simulink model "Y3Tiltrotor_sim3_INDI"  (R2025a)
settings: Solver=ode4  StartTime=0.0  StopTime=70  FixedStep=uavParam.sampleTime  RelTol=1e-3
PreLoadFcn:
  | filepath  = fileparts(get_param(bdroot, 'FileName'))
  | cd(filepath);
InitFcn:
  | Init_sim_INDI;
values from neighbouring files (symbols this model uses):
  control = struct    [Init_sim_INDI.m]
  env = struct    [InitData.m]
  flightState = struct    [Init_sim_INDI.m]
  FWSpeed0 = 15    [Init_sim_INDI.m]
  k_lpf_p = 50    [Init_sim_INDI.m]
  k_lpf_q = 80    [Init_sim_INDI.m]
  k_lpf_r = 5    [Init_sim_INDI.m]
  k_lpf_u = 10    [Init_sim_INDI.m]
  k_lpf_v = 1    [Init_sim_INDI.m]
  k_lpf_w = 50    [Init_sim_INDI.m]
  k_p = 5    [Init_sim_INDI.m]
  k_q = 20    [Init_sim_INDI.m]
  k_r = 1.5    [Init_sim_INDI.m]
  k_u = 0.5    [Init_sim_INDI.m]
  k_v = 0.5    [Init_sim_INDI.m]
  k_w = 2    [Init_sim_INDI.m]
  uavParam = struct    [InitData.m]
undefined symbols (not defined in the file or in its folder): ControlSampleTime, F, Light, MIL, Newton, Raphson
libraries: slpidlib x28, SignalEditorBlockLib x12, simulink x6, aerolibtransform2 x3, sharedtransform x3, robotcorelib x3, matrix_library x3, aerolibasang x2, aerolibutil x2, aerolibwind2 x2, shared6dof x1, aerolibatmos2 x1
(part 6 of 7)

== system Y3Tiltrotor_sim3_INDI/Y3 Tiltrotor Aircraft Model/Subsystem/Aerodynamic Forces and Moments/Compute Body Frame Aerodynamic Forces and Moments/Aerodynamic Forces and Moment Calculations/Subsystem1 ==
  AirData : Inport
  M_w : Inport  Port=2
  Bus Selector : BusSelector  OutputSignals=alpha,beta
  Direction Cosine Matrix Body to Wind : aerolibtransform2/Direction Cosine Matrix Body to Wind
  Mux1 : Mux  Inputs=2
  Product2 : Product  Multiplication=Matrix(*)  RndMeth=Zero
  Reshape1 : Reshape  OutputDimensionality=Column vector (2-D)
  Reshape2 : Reshape
  Transpose : Math  Operator=transpose  SignedPower=on
  M_b : Outport
  wires:
  AirData/1 -> Bus Selector/1
  Bus Selector/2 -> Mux1/2  "<beta>"
  Bus Selector/1 -> Mux1/1  "<alpha>"
  Direction Cosine Matrix Body to Wind/1 -> Transpose/1
  Reshape2/1 -> M_b/1
  Reshape1/1 -> Product2/2
  M_w/1 -> Reshape1/1
  Mux1/1 -> Direction Cosine Matrix Body to Wind/1
  Product2/1 -> Reshape2/1
  Transpose/1 -> Product2/1

== system Y3Tiltrotor_sim3_INDI/Y3 Tiltrotor Aircraft Model/Subsystem/Aerodynamic Forces and Moments/Compute Body Frame Aerodynamic Forces and Moments/Wind frame F& M/Lateral Channel ==
  note: 飞机没有尾翼，不需要考虑方向舵的影响，固定翼模态下做偏航运动时通过两个螺旋桨的推力差动来实现；其造成的侧力与偏航力矩在旋翼建模部分计算。
  beta : Inport
  dA : Inport  Port=2
  Bus Creator : BusCreator  Inputs=3
  CY : Subsystem
  Cl : Subsystem
  Cn : Subsystem
  Saturation2 : Saturate  UpperLimit=pi/2  LowerLimit=-pi/2
  固定翼模态使用 : Saturate  UpperLimit=41.5*pi/80  LowerLimit=-41.5*pi/80
  旋翼模态使用 : Saturate  UpperLimit=90*pi/80  LowerLimit=-90*pi/80
  Lateral : Outport  VectorParamsAs1DForOutWhenUnconnected=off
  wires:
  Cl/1(Cl) -> Bus Creator/2  "Cl"
  Cn/1(Cn) -> Bus Creator/3  "Cn"
  CY/1(CY) -> Bus Creator/1  "CY"
  Bus Creator/1 -> Lateral/1
  beta/1 -> 旋翼模态使用/1
  dA/1 -> Saturation2/1
  旋翼模态使用/1 -> Cn/1(beta), Cl/1(beta), CY/1(beta)
  Saturation2/1 -> Cn/2(dA), Cl/2(dA)

== system Y3Tiltrotor_sim3_INDI/Y3 Tiltrotor Aircraft Model/Subsystem/Aerodynamic Forces and Moments/Compute Body Frame Aerodynamic Forces and Moments/Wind frame F& M/Longitudinal Channel ==
  alpha : Inport
  dE : Inport  Port=2
  dA : Inport  Port=3
  Bus Creator : BusCreator  Inputs=3
  CD : Subsystem
  CL : Subsystem
  Cm : Subsystem
  Saturation1 : Saturate  UpperLimit=pi/2  LowerLimit=-pi/2
  Saturation2 : Saturate  UpperLimit=pi/2  LowerLimit=-pi/2
  固定翼模态使用 : Saturate  UpperLimit=18.4*pi/180  LowerLimit=-15*pi/180  LinearizeAsGain=off  ZeroCross=off
  旋翼模态使用 : Saturate  UpperLimit=90*pi/80  LowerLimit=-90*pi/80
  Longitudinal : Outport  VectorParamsAs1DForOutWhenUnconnected=off
  wires:
  Bus Creator/1 -> Longitudinal/1
  Cm/1(Cm) -> Bus Creator/3  "Cm"
  CL/1(CL) -> Bus Creator/2  "CL"
  CD/1(CD) -> Bus Creator/1  "CD"
  alpha/1 -> 旋翼模态使用/1
  dE/1 -> Saturation1/1
  Saturation1/1 -> Cm/2(dE), CL/2(dE), CD/2(dE)
  旋翼模态使用/1 -> Cm/1(alpha), CL/1(alpha), CD/1(alpha)
  dA/1 -> Saturation2/1
  Saturation2/1 -> CD/3(dA)

== system Y3Tiltrotor_sim3_INDI/Y3 Tiltrotor Aircraft Model/Subsystem/Aerodynamic Forces and Moments/Compute Body Frame Aerodynamic Forces and Moments/Wind frame F& M/Route coefficients ==
  Lateral : Inport
  Longitudinal : Inport  Port=2
  Bus Selector : BusSelector  OutputSignals=CY,Cl,Cn
  Bus Selector3 : BusSelector  OutputSignals=CD,CL,Cm
  <CD> : Outport
  <CY> : Outport  Port=2
  <CL> : Outport  Port=3
  <Cl> : Outport  Port=4
  <Cm> : Outport  Port=5
  <Cn> : Outport  Port=6
  wires:
  Bus Selector3/2 -> <CL>/1  "<CL>"
  Bus Selector/3 -> <Cn>/1  "<Cn>"
  Bus Selector/2 -> <Cl>/1  "<Cl>"
  Lateral/1 -> Bus Selector/1
  Bus Selector3/3 -> <Cm>/1  "<Cm>"
  Bus Selector3/1 -> <CD>/1  "<CD>"
  Longitudinal/1 -> Bus Selector3/1
  Bus Selector/1 -> <CY>/1  "<CY>"

== system Y3Tiltrotor_sim3_INDI/Subsystem/固定翼模态/高度-速度控制/定速模式/Subsystem1/Subsystem/InputConditioning_altitude ==
  Manual Vz_d : Inport
  Xe : Inport  Port=2
  Action Port : ActionPort  ActionPortLabel=case [ 1 ]:
  MATLAB Function : MATLAB Function  TreatAsAtomicUnit=on
  Selector : Selector  InputPortWidth=3  IndexOptions=Index vector (dialog)  Indices=3  OutputSizes=1
  manual_vz_cmd : Outport  VectorParamsAs1DForOutWhenUnconnected=off
  wires:
  MATLAB Function/1(vz_cmd) -> manual_vz_cmd/1
  Manual Vz_d/1 -> MATLAB Function/1(u)
  Selector/1 -> MATLAB Function/2(z_e)
  Xe/1 -> Selector/1

== system Y3Tiltrotor_sim3_INDI/Subsystem/固定翼模态/高度-速度控制/定速模式/Subsystem1/Subsystem/Subsystem ==
  Navigation Z : Inport
  Xe : Inport  Port=2
  Action Port : ActionPort  ActionPortLabel=case [ 0 ]:
  PID Controller1 : slpidlib/PID Controller  Controller=PID  Form=Parallel  TimeDomain=Continuous-time  UseExternalTs=off  SampleTime=ControlSampleTime  IntegratorMethod=Forward Euler  FilterMethod=Forward Euler  ControllerParametersSource=internal  P=control.FW.alt_P  I=control.FW.alt_I  UseKiTs=off  D=control.FW.alt_D  UseExternalDerivativeSource=off  N=100  UseFilter=on  TunerSelectOption=Transfer Function Based (PID Tuner App)  InitialConditionSource=internal  InitialConditionForIntegrator=0  InitialConditionForFilter=0  DifferentiatorICPrevScaledInput=0  ExternalReset=none  TrackingMode=off  Kt=1  LimitOutput=on  SatLimitsSource=internal  UpperSaturationLimit=control.maxClimbRate  LowerSaturationLimit=control.maxDescendRate  LinearizeAsGain=on  AntiWindupMode=clamping  Kb=1  LimitIntegrator=off  UpperIntegratorSaturationLimit=inf  LowerIntegratorSaturationLimit=-inf  POutMin=[]  POutMax=[]  IOutMin=[]  IOutMax=[]  DOutMin=[]  DOutMax=[]  NOutMin=[]  NOutMax=[]  SumOutMin=[]  SumOutMax=[]  SaturationOutMin=[]  SaturationOutMax=[]  PParamMin=[]  PParamMax=[]  IParamMin=[]  IParamMax=[]  DParamMin=[]  DParamMax=[]  NParamMin=[]  NParamMax=[]  KbParamMin=[]  KbParamMax=[]  KtParamMin=[]  KtParamMax=[]  KbOutMin=[]  KbOutMax=[]  KtOutMin=[]  KtOutMax=[]  IntegratorOutMin=[]  IntegratorOutMax=[]  FilterOutMin=[]  FilterOutMax=[]  SumI1OutMin=[]  SumI1OutMax=[]  SumI2OutMin=[]  SumI2OutMax=[]  SumI3OutMin=[]  SumI3OutMax=[]  SumI4OutMin=[]  SumI4OutMax=[]  SumDOutMin=[]  SumDOutMax=[]  DifferentiatorOutMin=[]  DifferentiatorOutMax=[]  FilterDiffOutCoefMin=[]  FilterDiffOutCoefMax=[]  ReciprocalOutMin=[]  ReciprocalOutMax=[]  SumDenOutMin=[]  SumDenOutMax=[]  SumNumOutMin=[]  SumNumOutMax=[]  DivideOutMin=[]  DivideOutMax=[]  UdiffTsProdOutMin=[]  UdiffTsProdOutMax=[]  NTsProdOutMin=[]  NTsProdOutMax=[]  UintegralTsProdOutMin=[]  UintegralTsProdOutMax=[]  UngainTsProdOutMin=[]  UngainTsProdOutMax=[]  ClampingZeroOutDataTypeStr=Inherit: Inherit via back propagation  ClampingZeroOutMin=[]  ClampingZeroOutMax=[]  FilterDenConstantOutDataTypeStr=Inherit: Inherit via back propagation  FilterDenConstantOutMin=[]  FilterDenConstantOutMax=[]  PCopyOutDataTypeStr=Inherit: Inherit via back propagation  PCopyOutMin=[]  PCopyOutMax=[]  NCopyOutDataTypeStr=Inherit: Inherit via back propagation  NCopyOutMin=[]  NCopyOutMax=[]  IntegratorContinuousStateAttributes=''  IntegratorStateMustResolveToSignalObject=off  IntegratorRTWStateStorageClass=Auto  FilterContinuousStateAttributes=''  FilterStateMustResolveToSignalObject=off  FilterRTWStateStorageClass=Auto  ParallelPVariant=InternalParameters  IdealPVariant=Disabled  IVariant=InternalParameters  DVariant=InternalParameters  IntegratorVariant=Continuous  SatVariant=Enabled  AWVariant=ContClampingParallel  PCopyVariant=Disabled  TRVariant=Disabled  FdbkBlocksVariant=Forward  IdealPFdbkVariant=Disabled  SatFdbkVariant=Disabled  DerivativeFilterVariant=ContFilter  NVariant=InternalParameters  NCopyVariant=Disabled  FilterICVariant=InternalICsFilter  IntegratorICVariant=InternalICs  ExternalResetVariant=Disabled  TRSumVariant=Passthrough  SumFdbkVariant=Disabled  SumVariant=Sum_PID  TsampFilterVariant=InternalTs  TsampNgainVariant=Passthrough  TsampIntegralVariant=Disabled_SignalSpec  ExternalSaturationOutDataTypeStr=Inherit: Same as second input  DerivativeSourceVariant=ErrorSignal  PreIntVariant=InternalPreInt
  Selector : Selector  InputPortWidth=3  IndexOptions=Index vector (dialog)  Indices=3  OutputSizes=1
  Sum : Sum  Inputs=|+-
  Unary Minus : UnaryMinus
  PID_vz_cmd : Outport
  wires:
  Unary Minus/1 -> Sum/2
  Selector/1 -> Unary Minus/1
  Xe/1 -> Selector/1
  Sum/1 -> PID Controller1/1
  PID Controller1/1 -> PID_vz_cmd/1
  Navigation Z/1 -> Sum/1

== system Y3Tiltrotor_sim3_INDI/Y3 Tiltrotor Aircraft Model/Subsystem/Aerodynamic Forces and Moments/Compute Body Frame Aerodynamic Forces and Moments/Wind frame F& M/Lateral Channel/CY ==
  beta : Inport
  CY(beta) : MATLAB Function  TreatAsAtomicUnit=on
  Gain : Gain  Gain=180/pi
  CY : Outport  VectorParamsAs1DForOutWhenUnconnected=off
  wires:
  CY(beta)/1(CY_beta) -> CY/1
  beta/1 -> Gain/1
  Gain/1 -> CY(beta)/1(beta)

== system Y3Tiltrotor_sim3_INDI/Y3 Tiltrotor Aircraft Model/Subsystem/Aerodynamic Forces and Moments/Compute Body Frame Aerodynamic Forces and Moments/Wind frame F& M/Lateral Channel/Cl ==
  beta : Inport
  dA : Inport  Port=2
  Cl(beta) : MATLAB Function  TreatAsAtomicUnit=on
  Cl(delta_a) : MATLAB Function  TreatAsAtomicUnit=on
  Gain : Gain  Gain=180/pi
  Gain1 : Gain  Gain=180/pi
  Gain2 : Gain
  Sum : Sum  Inputs=|++
  Cl : Outport  VectorParamsAs1DForOutWhenUnconnected=off
  wires:
  Gain/1 -> Cl(beta)/1(beta)
  beta/1 -> Gain/1
  dA/1 -> Gain1/1
  Sum/1 -> Gain2/1
  Gain1/1 -> Cl(delta_a)/1(delta_a)
  Cl(delta_a)/1(Cl1_delta_a) -> Sum/2
  Cl(beta)/1(Cl1_beta) -> Sum/1
  Gain2/1 -> Cl/1

== system Y3Tiltrotor_sim3_INDI/Y3 Tiltrotor Aircraft Model/Subsystem/Aerodynamic Forces and Moments/Compute Body Frame Aerodynamic Forces and Moments/Wind frame F& M/Lateral Channel/Cn ==
  beta : Inport
  dA : Inport  Port=2
  Cn(beta) : MATLAB Function  TreatAsAtomicUnit=on
  Cn(delta_a) : MATLAB Function  TreatAsAtomicUnit=on
  Gain : Gain  Gain=180/pi
  Gain1 : Gain  Gain=180/pi
  Gain2 : Gain
  Sum : Sum  Inputs=|++
  Cn : Outport  VectorParamsAs1DForOutWhenUnconnected=off
  wires:
  dA/1 -> Gain1/1
  beta/1 -> Gain/1
  Gain/1 -> Cn(beta)/1(beta)
  Sum/1 -> Gain2/1
  Cn(beta)/1(Cn_beta) -> Sum/1
  Gain1/1 -> Cn(delta_a)/1(delta_a)
  Cn(delta_a)/1(Cn_delta_a) -> Sum/2
  Gain2/1 -> Cn/1

== system Y3Tiltrotor_sim3_INDI/Y3 Tiltrotor Aircraft Model/Subsystem/Aerodynamic Forces and Moments/Compute Body Frame Aerodynamic Forces and Moments/Wind frame F& M/Longitudinal Channel/CD ==
  alpha : Inport
  dE : Inport  Port=2
  dA : Inport  Port=3
  CD(alpha) : MATLAB Function  TreatAsAtomicUnit=on
  CD(delta_a) : MATLAB Function  TreatAsAtomicUnit=on
  CD(delta_e) : MATLAB Function  TreatAsAtomicUnit=on
  Gain : Gain  Gain=180/pi
  Gain1 : Gain  Gain=180/pi
  Gain2 : Gain  Gain=180/pi
  Gain3 : Gain
  Gain4 : Gain
  Sum : Sum  Inputs=|+++
  CD : Outport  VectorParamsAs1DForOutWhenUnconnected=off
  wires:
  alpha/1 -> Gain/1
  CD(alpha)/1(CD_alpha) -> Gain4/1
  Gain/1 -> CD(alpha)/1(alpha)
  CD(delta_e)/1(CD_delta_e) -> Gain3/1
  Gain1/1 -> CD(delta_e)/1(delta_e)
  dE/1 -> Gain1/1
  dA/1 -> Gain2/1
  Gain2/1 -> CD(delta_a)/1(delta_a)
  CD(delta_a)/1(CD_delta_a) -> Sum/3
  Sum/1 -> CD/1
  Gain4/1 -> Sum/1
  Gain3/1 -> Sum/2

== system Y3Tiltrotor_sim3_INDI/Y3 Tiltrotor Aircraft Model/Subsystem/Aerodynamic Forces and Moments/Compute Body Frame Aerodynamic Forces and Moments/Wind frame F& M/Longitudinal Channel/CL ==
  alpha : Inport
  dE : Inport  Port=2
  CL(alpha) : MATLAB Function  TreatAsAtomicUnit=on
  CL(delta_e) : MATLAB Function  TreatAsAtomicUnit=on
  Gain : Gain  Gain=180/pi
  Gain1 : Gain  Gain=180/pi
  Gain2 : Gain
  Gain3 : Gain
  Sum : Sum  Inputs=|++
  CL : Outport  VectorParamsAs1DForOutWhenUnconnected=off
  wires:
  dE/1 -> Gain1/1
  alpha/1 -> Gain/1
  CL(delta_e)/1(CL_delta_e) -> Gain3/1
  CL(alpha)/1(CL_alpha) -> Gain2/1
  Gain/1 -> CL(alpha)/1(alpha)
  Gain1/1 -> CL(delta_e)/1(delta_e)
  Sum/1 -> CL/1
  Gain2/1 -> Sum/1
  Gain3/1 -> Sum/2

== system Y3Tiltrotor_sim3_INDI/Y3 Tiltrotor Aircraft Model/Subsystem/Aerodynamic Forces and Moments/Compute Body Frame Aerodynamic Forces and Moments/Wind frame F& M/Longitudinal Channel/Cm ==
  alpha : Inport
  dE : Inport  Port=2
  Cm(alpha) : MATLAB Function  TreatAsAtomicUnit=on
  Cm(delta_e) : MATLAB Function  TreatAsAtomicUnit=on
  Gain : Gain  Gain=180/pi
  Gain1 : Gain  Gain=180/pi
  Gain2 : Gain
  Sum : Sum  Inputs=|++
  修正系数 : Gain
  Cm : Outport  VectorParamsAs1DForOutWhenUnconnected=off
  wires:
  alpha/1 -> Gain/1
  Gain/1 -> Cm(alpha)/1(alpha)
  dE/1 -> Gain1/1
  Cm(alpha)/1(Cm_alpha) -> Sum/1
  Sum/1 -> Cm/1
  Cm(delta_e)/1(Cm_delta_e) -> 修正系数/1
  Gain1/1 -> Cm(delta_e)/1(delta_e)
  Gain2/1 -> Sum/2
  修正系数/1 -> Gain2/1

== matlab function Y3Tiltrotor_sim3_INDI/Y3 Tiltrotor Aircraft Model/Subsystem/Aerodynamic Forces and Moments/Compute Body Frame Aerodynamic Forces and Moments/Wind frame F& M/Longitudinal Channel/CD/CD(delta_a) ==
  data: delta_a input; CD_delta_a output
function CD_delta_a = fcn_CD_delta_a(delta_a)

    c1 = 0.069172;
    c2 = 0.000045;
    c3 = 0.063098;
    c4 = 0.057967;
    c5 = -0.926576;
    c6 = 6.280050;

    CD_delta_a = (1+tanh(c1*(45^2-delta_a.^2)))/(1+tanh(c1*45^2)).*(c2*delta_a.^2)...
            +(1-(1+tanh(c1*(45^2-delta_a.^2)))/(1+tanh(c1*45^2))).*(c3+c4*sin(c5*pi/180*delta_a+c6).^2);

end

== matlab function Y3Tiltrotor_sim3_INDI/Y3 Tiltrotor Aircraft Model/Subsystem/Aerodynamic Forces and Moments/Compute Body Frame Aerodynamic Forces and Moments/Wind frame F& M/Lateral Channel/Cl/Cl(delta_a) ==
  data: Cl1_delta_a output; delta_a input
function Cl1_delta_a = fcn_Cl1_delta_a(delta_a)

    c1 = 0.000009;
    c2 = 45;
    c3 = 0.112884;
    c4 = 1.470209;
    c5 = 0.194270;
    c6 = 6.811231;
    c7 = 9.431421;

    Cl1_delta_a = (1+tanh(c1*(c2^2-delta_a.^2)))/(1+tanh(c1*c2^2)).*(c3*sin(c4*pi/180*delta_a))...
        + (1-(1+tanh(c1*(c2^2-delta_a.^2)))/(1+tanh(c1*c2^2))).*(c5*sin(c6*pi/180*delta_a+c7));

end

== matlab function Y3Tiltrotor_sim3_INDI/Y3 Tiltrotor Aircraft Model/Subsystem/Aerodynamic Forces and Moments/Compute Body Frame Aerodynamic Forces and Moments/Wind frame F& M/Lateral Channel/Cn/Cn(delta_a) ==
  data: Cn_delta_a output; delta_a input
function Cn_delta_a = fcn_Cn_delta_a(delta_a)

    c1 = 953.946887;
    c2 = 52;
    c3 = -0.002040;
    c4 = 2.005880;
    c5 = -0.001991;
    c6 = 3.709436;
    c7 = 3.059122;

    Cn_delta_a = (1+tanh(c1*(c2^2-delta_a.^2)))/(1+tanh(c1*c2^2)).*(c3*sin(c4*pi/180*delta_a))...
        + (1-(1+tanh(c1*(c2^2-delta_a.^2)))/(1+tanh(c1*c2^2))).*(c5*sin(c6*pi/180*delta_a+c7));

end

== matlab function Y3Tiltrotor_sim3_INDI/Subsystem/固定翼模态/attitude control/Turn Coordinator/MATLAB Function ==
  data: rollSP input; rSP output; pitchSP input; airSpeed input
function rSP = fcn(rollSP, pitchSP, airSpeed)
    yawRateSP = tan(rollSP)*9.81/max(airSpeed,5);
    rSP = yawRateSP*cos(pitchSP)*cos(rollSP);
end

== matlab function Y3Tiltrotor_sim3_INDI/Subsystem/混控器/多旋翼混控/旋翼模态混控/MATLAB Function ==
  data: u_z input; w1 output; w2 output; w3 output; u_phi input; u_theta input
function [w1,w2,w3] = fcn(u_z,u_phi,u_theta)

    w1 = (1/(2+sqrt(3)))*u_z - (1/2)*u_phi + (sqrt(3)/(4+2*sqrt(3)))*u_theta;
    w2 = (1/(2+sqrt(3)))*u_z + (1/2)*u_phi + (sqrt(3)/(4+2*sqrt(3)))*u_theta;
    w3 = (sqrt(3)/(2+sqrt(3)))*u_z - (sqrt(3)/(2+sqrt(3)))*u_theta;

end

== matlab function Y3Tiltrotor_sim3_INDI/Subsystem/混控器/多旋翼混控/旋翼模态混控/MATLAB Function1 ==
  data: u_x input; Tilt1 output; Tilt2 output; u_psi input
function [Tilt1,Tilt2] = fcn(u_x,u_psi)

    Tilt1 = 1/2*(u_x - u_psi);
    Tilt2 = 1/2*(u_x + u_psi);

end

== matlab function Y3Tiltrotor_sim3_INDI/Subsystem/多旋翼模态/Multirotor altitude control/Subsystem/InputConditioning_altitude/MATLAB Function ==
  data: u input; vz_cmd output; z_e input
function vz_cmd = fcn(u,z_e)

    if z_e >= -0.001 && u < 0 
        vz_cmd = 0;
    else
        vz_cmd = u;
    end

end

== matlab function Y3Tiltrotor_sim3_INDI/Subsystem/混控器/多旋翼混控/旋翼模态混控/Multirotor Mixer2 (加上重力分量) ==
  data: u_z input; u_phi input; u_theta input; u_psi input; u_x input; w1 output; w2 output; w3 output; Tilt1 output; Tilt2 output; pitch input; roll input
function [w1,w2,w3,Tilt1,Tilt2] = fcn(u_z,u_phi,u_theta,u_psi,u_x,pitch,roll)
    
    m = 0.585;
    g = 9.80665;
    rho = 1.225;
    R = 0.765;
    k_1 = 19741.896106*2*pi/60;

    CT = 9.5883e-7;
    CQ = 1.4797e-8;
    R = 0.765;
    l1 = 0.13;
    l2 = 0.24;

    u_x_bar = u_x + m*g*sin(pitch)/(CT*rho*pi*R^4*k_1^2);
    u_z_bar = u_z - m*g*cos(roll)*cos(pitch)/(CT*rho*pi*R^4*k_1^2);

    k = (CQ*R)/CT;

    G = [0   1  0  1  1;
         k -l1 -k l1  0;
         0  l1  0 l1 -l2;
        -l1 -k l1  k  0;
         1  0   1  0  0];
    G_inv = inv(G);

    u = [u_z_bar,u_phi,u_theta,u_psi,u_x_bar]';
    u_act = G_inv*u;

    if u_act(2) == 0
        Tilt1_bar = 0;
    else
        Tilt1_bar = atan(u_act(1)/u_act(2));
    end
    if Tilt1_bar >= 45*pi/180
        Tilt1 = 45*pi/180;
    elseif Tilt1_bar <= -15*pi/180
        Tilt1 = -15*pi/180;
    else
        Tilt1 = Tilt1_bar;
    end

    if u_act(4) == 0
        Tilt2_bar = 0;
    else
        Tilt2_bar = atan(u_act(3)/u_act(4));
    end
    if Tilt2_bar >= 45*pi/180
        Tilt2 = 45*pi/180;
    elseif Tilt2_bar <= -15*pi/180
        Tilt2 = -15*pi/180;
    else
        Tilt2 = Tilt2_bar;
    end

    w1_bar = u_act(2)/cos(Tilt1);
    if w1_bar <= 0
        w1 = 0;
    else
        w1 = w1_bar;
    end

    w2_bar = u_act(4)/cos(Tilt2);
    if w2_bar <= 0
        w2 = 0;
    else
        w2 = w2_bar;
    end

    w3_bar = u_act(5);
    if w3_bar <= 0
        w3 = 0;
    else
        w3 = w3_bar;
    end

end

== matlab function Y3Tiltrotor_sim3_INDI/Subsystem/混控器/多旋翼混控/旋翼模态混控/Multirotor Mixer3 ==
  data: u_z input; u_phi input; u_theta input; u_psi input; u_x input; w1 output; w2 output; w3 output; Tilt1 output; Tilt2 output
function [w1,w2,w3,Tilt1,Tilt2] = fcn(u_z,u_phi,u_theta,u_psi,u_x)

    CT = 3.0123e-6;
    CQ = 4.6485e-8;
    R = 0.765;
    l1 = 0.13;
    l2 = 0.24;

    w1_bar = l2/(2*l1+2*l2)*u_z - 1/(2*l1)*u_phi + 1/(2*l1+2*l2)*u_theta;
    if w1_bar <= 0
        w1 = 0;
    else
        w1 = w1_bar;
    end

    w2_bar = l2/(2*l1+2*l2)*u_z + 1/(2*l1)*u_phi + 1/(2*l1+2*l2)*u_theta;
    if w2_bar <= 0
        w2 = 0;
    else
        w2 = w2_bar;
    end

    w3_bar = l1/(l1+l2)*u_z - 1/(l1+l2)*u_theta;
    if w3_bar <= 0
        w3 = 0;
    else
        w3 = w3_bar;
    end

    Tilt1_bar = (CQ*R/(2*CT*l1^2)*u_phi-1/(2*l1)*u_psi+0.5*u_x)/w1;
    if Tilt1_bar >= 45*pi/180
        Tilt1 = 45*pi/180;
    elseif Tilt1_bar <= -15*pi/180
        Tilt1 = -15*pi/180;
    elseif w1 == 0
        Tilt1 = 0;
    else
        Tilt1 = Tilt1_bar;
    end

    Tilt2_bar = (-CQ*R/(2*CT*l1^2)*u_phi+1/(2*l1)*u_psi+0.5*u_x)/w2;
    if Tilt2_bar >= 45*pi/180
        Tilt2 = 45*pi/180;
    elseif Tilt2_bar <= -15*pi/180
        Tilt2 = -15*pi/180;
    elseif w2 == 0
        Tilt2 = 0;
    else
        Tilt2 = Tilt2_bar;
    end

end

== matlab function Y3Tiltrotor_sim3_INDI/Subsystem/多旋翼模态/Multirotor XY control/Subsystem/InputConditioning_altitude/deadzone3 ==
  data: u input; y output
function y = fcn(u)
%Function description:
%  Control the range of the remote control input from RCMin to RCMax,which can be obtained from QGC. And set
%  a dead zone with a dead zone size of deadZone,the output y is normalized to 0~1.
RCMin = 1100;
RCMax = 1900;
RCMid = (RCMin + RCMax)/2;
deadZoneRate = 0.05;
deadZone = deadZoneRate*(RCMax - RCMin);
k = 1/(RCMax - RCMid - deadZone);
%Limiting
if(u < RCMin)
    u = RCMin;
elseif(u > RCMax)
    u = RCMax;
end
%dead zone and normalize
 if(u > RCMid + deadZone)
    y = (u-RCMid - deadZone)*k;
 elseif(u < RCMid - deadZone)
     y = (u - RCMid + deadZone)*k;
 else
     y = 0;
 end

 end

== matlab function Y3Tiltrotor_sim3_INDI/Subsystem/多旋翼模态/InputConditioning_stablelize/deadzone0 ==
  data: u input; y output
function y = fcn(u)
%Function description:
%  Control the range of the remote control input from RCMin to RCMax,which can be obtained from QGC. And set
%  a dead zone with a dead zone size of deadZone,the output y is normalized to 0~1.
RCMin = 1100;
RCMax = 1900;
RCMid = (RCMin + RCMax)/2;
deadZoneRate = 0.05;
deadZone = deadZoneRate*(RCMax - RCMin);
k = 1/(RCMax - RCMid - deadZone);
%Limiting
if(u < RCMin)
    u = RCMin;
elseif(u > RCMax)
    u = RCMax;
end
%dead zone and normalize
 if(u > RCMid + deadZone)
    y = (u-RCMid - deadZone)*k;
 elseif(u < RCMid - deadZone)
     y = (u - RCMid + deadZone)*k;
 else
     y = 0;
 end

 end

== matlab function Y3Tiltrotor_sim3_INDI/Subsystem/多旋翼模态/InputConditioning_stablelize/deadzone1 ==
  data: u input; y output
function y = fcn(u)
%Function description:
%  Control the range of the remote control input from RCMin to RCMax,which can be obtained from QGC. And set
%  a dead zone with a dead zone size of deadZone,the output y is normalized to 0~1.
RCMin = 1100;
RCMax = 1900;
RCMid = (RCMin + RCMax)/2;
deadZoneRate = 0.05;
deadZone = deadZoneRate*(RCMax - RCMin);
k = 1/(RCMax - RCMid - deadZone);
%Limiting
if(u < RCMin)
    u = RCMin;
elseif(u > RCMax)
    u = RCMax;
end
%dead zone and normalize
 if(u > RCMid + deadZone)
    y = (u-RCMid - deadZone)*k;
 elseif(u < RCMid - deadZone)
     y = (u - RCMid + deadZone)*k;
 else
     y = 0;
 end

 end

== matlab function Y3Tiltrotor_sim3_INDI/Subsystem/多旋翼模态/InputConditioning_stablelize/deadzone2 ==
  data: u input; y output
function y = fcn(u)
%Function description:
%  Control the range of the remote control input from RCMin to RCMax,which can be obtained from QGC. And set
%  a dead zone with a dead zone size of deadZone,the output y is normalized to 0~1.
RCMin = 1100;
RCMax = 1900;
RCMid = (RCMin + RCMax)/2;
deadZoneRate = 0.05;
deadZone = deadZoneRate*(RCMax - RCMin);
k = 1/(RCMax - RCMid - deadZone);
%Limiting
if(u < RCMin)
    u = RCMin;
elseif(u > RCMax)
    u = RCMax;
end
%dead zone and normalize
 if(u > RCMid + deadZone)
    y = (u-RCMid - deadZone)*k;
 elseif(u < RCMid - deadZone)
     y = (u - RCMid + deadZone)*k;
 else
     y = 0;
 end

 end

== matlab function Y3Tiltrotor_sim3_INDI/Subsystem/多旋翼模态/InputConditioning_stablelize/deadzone3 ==
  data: u input; y output
function y = fcn(u)
%Function description:
%  Control the range of the remote control input from RCMin to RCMax,which can be obtained from QGC. And set
%  a dead zone with a dead zone size of deadZone,the output y is normalized to 0~1.
RCMin = 1100;
RCMax = 1900;
RCMid = (RCMin + RCMax)/2;
deadZoneRate = 0.05;
deadZone = deadZoneRate*(RCMax - RCMin);
k = 1/(RCMax - RCMid - deadZone);
%Limiting
if(u < RCMin)
    u = RCMin;
elseif(u > RCMax)
    u = RCMax;
end
%dead zone and normalize
 if(u > RCMid + deadZone)
    y = (u-RCMid - deadZone)*k;
 elseif(u < RCMid - deadZone)
     y = (u - RCMid + deadZone)*k;
 else
     y = 0;
 end

 end

== matlab function Y3Tiltrotor_sim3_INDI/Subsystem/多旋翼模态/Multirotor attitude control (INDI)/Subsystem/Subsystem1/MATLAB Function ==
  settings: updateMethod=DISCRETE
  data: yaw_rate_d output; yaw_rate_desired input; yaw input; yaw_rate input; yaw_d output
function [yaw_rate_d, yaw_d] = fcn_yaw(yaw_rate_desired, yaw, yaw_rate)
% 偏航通道控制函数（与高度通道相同逻辑）
% Input:
%   yaw_rate_desired: 期望的偏航角速度（遥控器指令）
%   yaw: 当前偏航角
%   yaw_rate: 当前偏航角速度
% Output:
%   yaw_rate_d: 期望偏航角速度（传递给控制器）
%   yaw_d: 期望偏航角（传递给控制器）

persistent yaw1;
if isempty(yaw1)
    yaw1 = yaw;
end

persistent hold_yaw_flag;
if isempty(hold_yaw_flag)
    hold_yaw_flag = 0;
end

% 判断是否满足偏航锁定条件
% 条件1：期望偏航角速度很小（遥控器在中位）
% 条件2：当前偏航角速度也很小（飞行器稳定）
if abs(yaw_rate_desired) < 0.001 && abs(yaw_rate) < 0.1
    hold_yaw = 1;  % 满足锁定条件
else
    hold_yaw = 0;  % 不满足锁定条件
    hold_yaw_flag = 0;  % 重置锁定标志
end

% 首次满足锁定条件时，记录当前偏航角
% 遥控器回中且飞行器稳定时，锁定当前偏航角
if (hold_yaw > 0.5) && (hold_yaw_flag < 0.5)
    yaw1 = yaw;            % 记录当前偏航角作为锁定角度
    hold_yaw_flag = 1;     % 设置锁定标志
end

% 遥控器偏离中位，退出锁定模式
% 期望偏航角跟随当前偏航角
if hold_yaw < 0.5
    yaw1 = yaw;            % 期望偏航角 = 当前偏航角
    hold_yaw_flag = 0;     % 清除锁定标志
end

% 输出
yaw_rate_d = yaw_rate_desired;  % 直接传递期望角速度
yaw_d = yaw1;                   % 输出计算得到的期望偏航角

== matlab function Y3Tiltrotor_sim3_INDI/Subsystem/多旋翼模态/Multirotor altitude control/Subsystem/InputConditioning_altitude/deadzone3 ==
  data: u input; y output
function y = fcn(u)
%Function description:
%  Control the range of the remote control input from RCMin to RCMax,which can be obtained from QGC. And set
%  a dead zone with a dead zone size of deadZone,the output y is normalized to 0~1.
RCMin = 1100;
RCMax = 1900;
RCMid = (RCMin + RCMax)/2;
deadZoneRate = 0.05;
deadZone = deadZoneRate*(RCMax - RCMin);
k = 1/(RCMax - RCMid - deadZone);
%Limiting
if(u < RCMin)
    u = RCMin;
elseif(u > RCMax)
    u = RCMax;
end
%dead zone and normalize
 if(u > RCMid + deadZone)
    y = (u-RCMid - deadZone)*k;
 elseif(u < RCMid - deadZone)
     y = (u - RCMid + deadZone)*k;
 else
     y = 0;
 end

 end

== matlab function Y3Tiltrotor_sim3_INDI/Joystick and Waypoint Design/MATLAB Function2 ==
  data: ch5 input; control_mode output
function control_mode  = fcn(ch5)
%Function description:
%  Map the remote control CH5 channel to control mode
%input:
%  ch5: Remote control CH5 channel input
%  control_mode: Custom control mode
%  0: stablelize mode；1: height control mode; 2: position control mode
if ch5 < 1400
    control_mode = int8(0);
elseif ch5 < 1600
    control_mode = int8(1);
else
    control_mode = int8(2);
end

== matlab function Y3Tiltrotor_sim3_INDI/Subsystem/多旋翼模态/Multirotor XY control/Subsystem3/InputConditioning_altitude/deadzone3 ==
  data: u input; y output
function y = fcn(u)
%Function description:
%  Control the range of the remote control input from RCMin to RCMax,which can be obtained from QGC. And set
%  a dead zone with a dead zone size of deadZone,the output y is normalized to 0~1.
RCMin = 1100;
RCMax = 1900;
RCMid = (RCMin + RCMax)/2;
deadZoneRate = 0.05;
deadZone = deadZoneRate*(RCMax - RCMin);
k = 1/(RCMax - RCMid - deadZone);
%Limiting
if(u < RCMin)
    u = RCMin;
elseif(u > RCMax)
    u = RCMax;
end
%dead zone and normalize
 if(u > RCMid + deadZone)
    y = (u-RCMid - deadZone)*k;
 elseif(u < RCMid - deadZone)
     y = (u - RCMid + deadZone)*k;
 else
     y = 0;
 end

 end

== matlab function Y3Tiltrotor_sim3_INDI/Subsystem/多旋翼模态/MATLAB Function ==
  data: u_vy input; roll_d output
function roll_d = fcn(u_vy)

    m = 0.585;
    g = 9.81;
    
    roll_d = u_vy/(m*g);

end

== matlab function Y3Tiltrotor_sim3_INDI/Subsystem/混控器/多旋翼混控/旋翼模态混控/Multirotor Mixer1 ==
  data: u_z input; u_phi input; u_theta input; u_psi input; u_x input; w1 output; w2 output; w3 output; Tilt1 output; Tilt2 output
function [w1,w2,w3,Tilt1,Tilt2] = fcn(u_z,u_phi,u_theta,u_psi,u_x)

    CT = 3.0123e-6;
    CQ = 4.6485e-8;
    R = 0.765;
    l = 0.2;

    if (1/(2+sqrt(3))*u_z-0.5*u_phi+sqrt(3)/(4+2*sqrt(3))*u_theta) == 0
        Tilt1_bar = 0;
    else
        Tilt1_bar = atan((CQ*R/(CT*l)*u_phi-1/l*u_psi+0.5*u_x)/(1/(2+sqrt(3))*u_z-0.5*u_phi+sqrt(3)/(4+2*sqrt(3))*u_theta));
    end
    if Tilt1_bar >= 45*pi/180
        Tilt1 = 45*pi/180;
    elseif Tilt1_bar <= -15*pi/180
        Tilt1 = -15*pi/180;
    else
        Tilt1 = Tilt1_bar;
    end

    if (1/(2+sqrt(3))*u_z+0.5*u_phi+sqrt(3)/(4+2*sqrt(3))*u_theta) == 0
        Tilt2_bar = 0;
    else
        Tilt2_bar = atan((-CQ*R/(CT*l)*u_phi+1/l*u_psi+0.5*u_x)/(1/(2+sqrt(3))*u_z+0.5*u_phi+sqrt(3)/(4+2*sqrt(3))*u_theta));
    end
    if Tilt2_bar >= 45*pi/180
        Tilt2 = 45*pi/180;
    elseif Tilt2_bar <= -15*pi/180
        Tilt2 = -15*pi/180;
    else
        Tilt2 = Tilt2_bar;
    end

    w1 = ((1/(2+sqrt(3)))*u_z - (1/2)*u_phi + (sqrt(3)/(4+2*sqrt(3)))*u_theta)/cos(Tilt1);
    w2 = ((1/(2+sqrt(3)))*u_z + (1/2)*u_phi + (sqrt(3)/(4+2*sqrt(3)))*u_theta)/cos(Tilt2);
    w3 = (sqrt(3)/(2+sqrt(3)))*u_z - (sqrt(3)/(2+sqrt(3)))*u_theta;

end

== matlab function Y3Tiltrotor_sim3_INDI/Subsystem/混控器/多旋翼混控/旋翼模态混控/Multirotor Mixer4 (对应论文) ==
  data: u_z input; u_phi input; u_theta input; u_psi input; u_x input; w1 output; w2 output; w3 output; Tilt1 output; Tilt2 output
function [w1,w2,w3,Tilt1,Tilt2] = fcn(u_z,u_phi,u_theta,u_psi,u_x)
    
    CT = 9.5883e-7;
    CQ = 1.4797e-8;
    R = 0.765;
    l1 = 0.13;
    l2 = 0.24;

    k = (CQ*R)/CT;

    G = [0   1  0  1  1;
         k -l1 -k l1  0;
         0  l1  0 l1 -l2;
        -l1 -k l1  k  0;
         1  0   1  0  0];
    G_inv = inv(G);

    u = [u_z,u_phi,u_theta,u_psi,u_x]';
    u_act = G_inv*u;

    if u_act(2) == 0
        Tilt1_bar = 0;
    else
        Tilt1_bar = atan(u_act(1)/u_act(2));
    end
    if Tilt1_bar >= 45*pi/180
        Tilt1 = 45*pi/180;
    elseif Tilt1_bar <= -15*pi/180
        Tilt1 = -15*pi/180;
    else
        Tilt1 = Tilt1_bar;
    end

    if u_act(4) == 0
        Tilt2_bar = 0;
    else
        Tilt2_bar = atan(u_act(3)/u_act(4));
    end
    if Tilt2_bar >= 45*pi/180
        Tilt2 = 45*pi/180;
    elseif Tilt2_bar <= -15*pi/180
        Tilt2 = -15*pi/180;
    else
        Tilt2 = Tilt2_bar;
    end

    w1_bar = u_act(2)/cos(Tilt1);
    if w1_bar <= 0
        w1 = 0;
    else
        w1 = w1_bar;
    end

    w2_bar = u_act(4)/cos(Tilt2);
    if w2_bar <= 0
        w2 = 0;
    else
        w2 = w2_bar;
    end

    w3_bar = u_act(5);
    if w3_bar <= 0
        w3 = 0;
    else
        w3 = w3_bar;
    end

end

== matlab function Y3Tiltrotor_sim3_INDI/Joystick and Waypoint Design/MATLAB Function ==
  data: t input; x_ref output; y_ref output; z_ref output; psi_ref output; theta_ref output
function [x_ref, y_ref, z_ref, psi_ref, theta_ref] = generate_trajectory_fixed_yaw(t)
% 生成8字形轨迹（固定偏航角）
% 输入：当前时间 t（秒）
% 输出：期望位置x,y,z和偏航角psi

% 参数定义
T_takeoff = 20;     % 起飞阶段持续时间（秒）
H_cruise = 50;      % 巡航高度（米）
A = 10;              % 8字形x方向振幅（米）
B = 8;              % 8字形y方向振幅（米）
omega = 0.2;        % 角频率（rad/s）
circles = 3;         % 8字形飞行圈数
T_circle = 2*pi/omega; % 单圈周期（秒）
T_cruise = circles * T_circle; % 巡航总时间
T_land = 20;         % 降落阶段持续时间（秒）

% 计算任务总时间和各阶段时间点
T_total = T_takeoff + T_cruise + T_land;
t_cruise_start = T_takeoff;
t_land_start = T_takeoff + T_cruise;

% 偏航角固定为0（朝北）
psi_fixed = 0;

    % 起飞阶段（0 ≤ t < T_takeoff）
    if t < T_takeoff
        % 垂直起飞
        x_ref = 0;
        y_ref = 0;
        z_ref = (t / T_takeoff) * H_cruise;  % 线性上升
        psi_ref = psi_fixed;
        theta_ref = 0;
        
    elseif t < t_land_start
        % 8字形轨迹阶段
        t_cruise = t - t_cruise_start;
        
        % 8字形参数方程（Lemniscate of Bernoulli）
        % 使用改进的8字形方程，避免奇点
        theta = omega * t_cruise;
        
        % 方法1：使用椭圆8字形
        x_ref = A * sin(theta);
        y_ref = B * sin(2 * theta) / 2;
        
        % 方法2：使用更平滑的8字形（可选）
        % r = sqrt(cos(2*theta) + sqrt(1.1 - sin(2*theta)^2));
        % x_ref = A * r * cos(theta);
        % y_ref = B * r * sin(theta);
        
        z_ref = H_cruise;
        psi_ref = psi_fixed;
        theta_ref = 0;
    
    elseif t < T_total
        % 计算降落阶段的时间
        t_land = t - t_land_start;
        tau = t_land / T_land;
        
        % 平滑过渡到降落（使用五次多项式）
        % 从8字形的结束位置平滑回到原点
        theta_end = omega * T_cruise;
        x_end = A * sin(theta_end);
        y_end = B * sin(2 * theta_end) / 2;
        
        % 位置从8字形结束点平滑回到原点
        x_ref = x_end * (1 - tau);
        y_ref = y_end * (1 - tau);
        
        % 高度平滑下降（从H_cruise到0）
        z_ref = H_cruise * (1 - tau);
        psi_ref = psi_fixed;
        theta_ref = 0;
    
    else
        x_ref = 0;
        y_ref = 0;
        z_ref = 0;
        psi_ref = psi_fixed;
        theta_ref = 0;
    end



end

== matlab function Y3Tiltrotor_sim3_INDI/Subsystem/固定翼模态/InputConditioning_stablelize/deadzone0 ==
  data: u input; y output
function y = fcn(u)
%Function description:
%  Control the range of the remote control input from RCMin to RCMax,which can be obtained from QGC. And set
%  a dead zone with a dead zone size of deadZone,the output y is normalized to 0~1.
RCMin = 1100;
RCMax = 1900;
RCMid = (RCMin + RCMax)/2;
deadZoneRate = 0.05;
deadZone = deadZoneRate*(RCMax - RCMin);
k = 1/(RCMax - RCMid - deadZone);
%Limiting
if(u < RCMin)
    u = RCMin;
elseif(u > RCMax)
    u = RCMax;
end
%dead zone and normalize
 if(u > RCMid + deadZone)
    y = (u-RCMid - deadZone)*k;
 elseif(u < RCMid - deadZone)
     y = (u - RCMid + deadZone)*k;
 else
     y = 0;
 end

 end

== matlab function Y3Tiltrotor_sim3_INDI/Y3 Tiltrotor Aircraft Model/Subsystem/Aerodynamic Forces and Moments/Compute Body Frame Aerodynamic Forces and Moments/Wind frame F& M/Longitudinal Channel/CL/CL(delta_e) ==
  data: delta_e input; CL_delta_e output
function CL_delta_e = fcn_CL_delta_e(delta_e)

    c1 = 0.000343;
    c2 = 47.4;
    c3 = -11.336446;
    c4 = -0.081703;
    c5 = -0.548177;
    c6 = -0.772571;
    c7 = 25.051196;

    CL_delta_e = (1+tanh(c1*(c2^2-delta_e.^2)))/(1+tanh(c1*c2^2)).*(c3*sin(c4*pi/180*delta_e))...
            +(1-(1+tanh(c1*(c2^2-delta_e.^2)))/(1+tanh(c1*c2^2))).*(c5*sin(c6*pi/180*delta_e+c7));
    
end

== matlab function Y3Tiltrotor_sim3_INDI/Subsystem/固定翼模态/InputConditioning_stablelize/deadzone1 ==
  data: u input; y output
function y = fcn(u)
%Function description:
%  Control the range of the remote control input from RCMin to RCMax,which can be obtained from QGC. And set
%  a dead zone with a dead zone size of deadZone,the output y is normalized to 0~1.
RCMin = 1100;
RCMax = 1900;
RCMid = (RCMin + RCMax)/2;
deadZoneRate = 0.05;
deadZone = deadZoneRate*(RCMax - RCMin);
k = 1/(RCMax - RCMid - deadZone);
%Limiting
if(u < RCMin)
    u = RCMin;
elseif(u > RCMax)
    u = RCMax;
end
%dead zone and normalize
 if(u > RCMid + deadZone)
    y = (u-RCMid - deadZone)*k;
 elseif(u < RCMid - deadZone)
     y = (u - RCMid + deadZone)*k;
 else
     y = 0;
 end

 end

== matlab function Y3Tiltrotor_sim3_INDI/Subsystem/固定翼模态/InputConditioning_stablelize/deadzone2 ==
  data: u input; y output
function y = fcn(u)
%Function description:
%  Control the range of the remote control input from RCMin to RCMax,which can be obtained from QGC. And set
%  a dead zone with a dead zone size of deadZone,the output y is normalized to 0~1.
RCMin = 1100;
RCMax = 1900;
RCMid = (RCMin + RCMax)/2;
deadZoneRate = 0.05;
deadZone = deadZoneRate*(RCMax - RCMin);
k = 1/(RCMax - RCMid - deadZone);
%Limiting
if(u < RCMin)
    u = RCMin;
elseif(u > RCMax)
    u = RCMax;
end
%dead zone and normalize
 if(u > RCMid + deadZone)
    y = (u-RCMid - deadZone)*k;
 elseif(u < RCMid - deadZone)
     y = (u - RCMid + deadZone)*k;
 else
     y = 0;
 end

 end

== matlab function Y3Tiltrotor_sim3_INDI/Subsystem/固定翼模态/InputConditioning_stablelize/deadzone3 ==
  data: u input; y output
function y = fcn(u)
%Function description:
%  Control the range of the remote control input from RCMin to RCMax,which can be obtained from QGC. And set
%  a dead zone with a dead zone size of deadZone,the output y is normalized to 0~1.
RCMin = 1000;
RCMax = 2000;
RCMid = (RCMin + RCMax)/2;
deadZoneRate = 0.05;
deadZone = deadZoneRate*(RCMax - RCMin);
k = 1/(RCMax - RCMid - deadZone);
%Limiting
if(u < RCMin)
    u = RCMin;
elseif(u > RCMax)
    u = RCMax;
end
%dead zone and normalize
 if(u > RCMid + deadZone)
    y = (u-RCMid - deadZone)*k;
 elseif(u < RCMid - deadZone)
     y = (u - RCMid + deadZone)*k;
 else
     y = 0;
 end

 end

== matlab function Y3Tiltrotor_sim3_INDI/Subsystem/固定翼模态/InputConditioning_altitude/deadzone3 ==
  data: u input; y output
function y = fcn(u)
%Function description:
%  Control the range of the remote control input from RCMin to RCMax,which can be obtained from QGC. And set
%  a dead zone with a dead zone size of deadZone,the output y is normalized to 0~1.
RCMin = 1100;
RCMax = 1900;
RCMid = (RCMin + RCMax)/2;
deadZoneRate = 0.05;
deadZone = deadZoneRate*(RCMax - RCMin);
k = 1/(RCMax - RCMid - deadZone);
%Limiting
if(u < RCMin)
    u = RCMin;
elseif(u > RCMax)
    u = RCMax;
end
%dead zone and normalize
 if(u > RCMid + deadZone)
    y = (u-RCMid - deadZone)*k;
 elseif(u < RCMid - deadZone)
     y = (u - RCMid + deadZone)*k;
 else
     y = 0;
 end

 end

== matlab function Y3Tiltrotor_sim3_INDI/Subsystem/固定翼模态/InputConditioning_speed/deadzone3 ==
  data: u input; y output
function y = fcn(u)
%Function description:
%  Control the range of the remote control input from RCMin to RCMax,which can be obtained from QGC. And set
%  a dead zone with a dead zone size of deadZone,the output y is normalized to 0~1.
RCMin = 1100;
RCMax = 1900;
RCMid = (RCMin + RCMax)/2;
deadZoneRate = 0.05;
deadZone = deadZoneRate*(RCMax - RCMin);
k = 1/(RCMax - RCMid - deadZone);
%Limiting
if(u < RCMin)
    u = RCMin;
elseif(u > RCMax)
    u = RCMax;
end
%dead zone and normalize
 if(u > RCMid + deadZone)
    y = (u-RCMid - deadZone)*k;
 elseif(u < RCMid - deadZone)
     y = (u - RCMid + deadZone)*k;
 else
     y = 0;
 end

 end

== matlab function Y3Tiltrotor_sim3_INDI/Subsystem/固定翼模态/高度-速度控制/定速模式/TECS/MATLAB Function ==
  data: Airspeed input; V output
function V = fcn(Airspeed)

    if abs(Airspeed) <= 0.001
        V = 0.001;
    else
        V = Airspeed;
    end

end

== matlab function Y3Tiltrotor_sim3_INDI/Subsystem/固定翼模态/高度-速度控制/定速模式/Subsystem1/Subsystem/InputConditioning_altitude/MATLAB Function ==
  data: u input; vz_cmd output; z_e input
function vz_cmd = fcn(u,z_e)

    if z_e >= -0.001 && u < 0 
        vz_cmd = 0;
    else
        vz_cmd = u;
    end

end

== matlab function Y3Tiltrotor_sim3_INDI/Subsystem/固定翼模态/高度-速度控制/定高模式/Subsystem/InputConditioning_altitude/MATLAB Function ==
  data: u input; vz_cmd output; z_e input
function vz_cmd = fcn(u,z_e)

    if z_e >= -0.001 && u < 0 
        vz_cmd = 0;
    else
        vz_cmd = u;
    end

end

== matlab function Y3Tiltrotor_sim3_INDI/Subsystem/多旋翼模态/Multirotor attitude control (INDI)/INDI in vector form/r_测量噪声/MATLAB Function1 ==
  data: t input; r_mea output; r input; r_noise input
function r_mea = fcn(t,r,r_noise)


    if  t>30 && t<41
        r_mea = r_noise;
    else
        r_mea = r;
    end


end

== matlab function Y3Tiltrotor_sim3_INDI/Y3 Tiltrotor Aircraft Model/Subsystem/Aerodynamic Forces and Moments/Compute Body Frame Aerodynamic Forces and Moments/Wind frame F& M/Longitudinal Channel/CL/CL(alpha) ==
  data: CL_alpha output; alpha input
function CL_alpha = piecewise_CL_alpha(alpha)

    c1 = 51.38;
    c2 = 18.4;
    c3 = 0.106096;
    c4 = -0.999417;
    c5 = -3.039833;
    c6 = -0.864898;
    c7 = 0.956252;
    c8 = -1.573247;
    c9 = 5.019980;
    c10 = 14.998103;
    c11 = 0.619631;
    c12 = 1.474257;
    c13 = 5.709070;

    CL_alpha = zeros(size(alpha));

    idx_pos = alpha >= 0;
    if any(idx_pos)
        alpha_pos = alpha(idx_pos);
        CL_alpha(idx_pos) = (1+tanh(c1*(c2^2-alpha_pos.^2)))/(1+tanh(c1*c2^2)).*(c3+c4*sin(c5*pi/180*alpha_pos))...
            +(1-(1+tanh(c1*(c2^2-alpha_pos.^2)))/(1+tanh(c1*c2^2))).*(c6*sin(c7*pi/180*alpha_pos+c8));
    end
    
    idx_neg = alpha < 0;
    if any(idx_neg)
        alpha_neg = alpha(idx_neg);
        CL_alpha(idx_neg) = (1+tanh(c9*(c10^2-alpha_neg.^2)))/(1+tanh(c9*c10^2)).*(c3+c4*sin(c5*pi/180*alpha_neg))...
            +(1-(1+tanh(c9*(c10^2-alpha_neg.^2)))/(1+tanh(c9*c10^2))).*(c11*sin(c12*pi/180*alpha_neg+c13));
    end

end

== matlab function Y3Tiltrotor_sim3_INDI/Joystick and Waypoint Design/MATLAB Function1 ==
  data: t input; x_ref output; y_ref output; z_ref output; psi_ref output; theta_ref output
function [x_ref, y_ref, z_ref, psi_ref, theta_ref] = generate_trajectory_pure_8(t)
% 生成简化的8字形轨迹（无起降，10秒后开始飞行，仅飞一圈）
% 特性：初始高度-75m，前10s悬停，10s后开始飞8字，飞完一圈后原地悬停。
%       俯仰角恒为0，偏航角在飞行期间始终对准前进方向。
% 输入：当前时间 t（秒）
% 输出：期望位置 x,y,z 以及期望偏航角 psi, 俯仰角 theta

% 参数定义
H_cruise = 75;     % 始终保持的巡航高度（米）
A = 10;             % 8字形x方向振幅（米）
B = 8;              % 8字形y方向振幅（米）
omega = pi/20;        % 角频率（rad/s）
circles = 2;        % 飞行圈数设为 2 圈

T_start = 20;                  % 8字形飞行开始时间（秒）
T_circle = 2*pi/omega;         % 飞一圈所需的时间（秒）
T_end = T_start + circles*T_circle;    % 8字形飞行结束时间（秒）

% 提前计算8字形起点的切线方向角（t_cruise = 0 时，vx = A*omega, vy = B*omega）
psi_hover = atan2(B*omega, A*omega);

    % 阶段 1：前 10 秒悬停阶段
    if t < T_start
        x_ref = 0;
        y_ref = 0;
        z_ref = H_cruise;
        psi_ref = psi_hover;  % 提前对准8字形起点的航向，防止10秒时航向突变
        theta_ref = 0;        % 俯仰角始终为0
        
    % 阶段 2：8 字形飞行阶段（仅飞一圈）
    elseif t < T_end
        % 计算8字形轨迹的有效巡航时间
        t_cruise = t - T_start;
        theta = omega * t_cruise;
        
        % 8字形位置方程
        x_ref = A * sin(theta);
        y_ref = B * sin(2 * theta) / 2;
        
        % 对位置求导得到速度矢量，用于计算航向角
        vx = A * omega * cos(theta);
        vy = B * omega * cos(2 * theta);
        
        z_ref = H_cruise;
        psi_ref = atan2(vy, vx);  % 偏航角时刻对准前进方向
        theta_ref = 0;            % 俯仰角始终为0
    
    % 阶段 3：飞行结束后的原地悬停阶段
    else
        % 一圈结束时 theta = 2*pi，轨迹刚好完美回到原点 [0, 0]
        x_ref = 0;
        y_ref = 0;
        z_ref = H_cruise;
        psi_ref = psi_hover;      % 回到起点，航向也刚好恢复到初始切线方向
        theta_ref = 0;            % 俯仰角始终为0
    end
end

== matlab function Y3Tiltrotor_sim3_INDI/Subsystem/多旋翼模态/Multirotor attitude control (INDI)/Subsystem/Subsystem/MATLAB Function ==
  data: e_yaw_old input; e_yaw_new output
function e_yaw_new = fcn(e_yaw_old)

    e_yaw_new = mod(e_yaw_old+pi,2*pi) - pi;

end

== matlab function Y3Tiltrotor_sim3_INDI/Y3 Tiltrotor Aircraft Model/Subsystem/MATLAB Function ==
  data: t input; dv output
function dv = fcn(t)

T = t-(41);
% 
%     if t < 10+(pi/0.2)
%         dv = [0;0;0];
%     else
%         dv = [0.4+0.8*sin(3*T);0;0];
%         % dv = [0;0;0];
%     end


    % if t>5  && t<=10+(pi/0.2)
    %     dv = [0.4+0.5*sin(3*(t-5));0;0.5*cos(5*(t-5))];
    % else
    %     dv = [0;0;0];
    % end

    if t < (41)
        dv = [0;0;0];
    else
        % dv = [0.4+0.5*sin(3*(T));0.2;0.3*cos(5*(T))];
        % dv = [0;0;0];
        % dv = [0.4+0.5*sin(3*(T));0.2;0.3*cos(5*(T))];
        % dv = [-0.4;0.3*sin(2*T);0.3*cos(5*(T))];
        % dv = [-0.5+0.4*sin(3*(T));0;0.6*cos(5*(T))];
        dv = [-0.5+0.4*sin(3*(T));0.3*sin(2*T);0.8*cos(2*(T))];
    end

    
end

== matlab function Y3Tiltrotor_sim3_INDI/Y3 Tiltrotor Aircraft Model/Subsystem/MATLAB Function1 ==
  data: t input; dw output
function dw = fcn(t)

% T = t-10+(pi/2/0.2);
% 
%     if t < 10+(pi/0.2)
%         dv = [0;0;0];
%     else
%         dv = [0.4+0.8*sin(3*T);0;0];
%         % dv = [0;0;0];
%     end


    % if t>5  && t<=10+(pi/0.2)
    %     dw = [0;0.2*sin(2*(t-5));0.03*sin(1*(t-5))];
    % else
    %     dw = [0;0;0];
    % end

T = t-(41);

    if t < (41)
        dw = [0;0;0];
    else
        % dw = [0;0.2*sin(2*(T));0.1*sin(1*(T))];
        dw = [0;0.2*sin(1*(T));0.05*sin(0.3*(T))];
        % dw = [0;0;0];
    end


end

== matlab function Y3Tiltrotor_sim3_INDI/Subsystem/多旋翼模态/Multirotor attitude control (INDI)/INDI in vector form/q_测量噪声/MATLAB Function1 ==
  data: t input; r_mea output; r input; r_noise input
function r_mea = fcn(t,r,r_noise)


    if  t>30 && t<41
        r_mea = r_noise;
    else
        r_mea = r;
    end


end

== matlab function Y3Tiltrotor_sim3_INDI/Subsystem/多旋翼模态/Multirotor attitude control (INDI)/INDI in vector form/p_测量噪声/MATLAB Function1 ==
  data: t input; r_mea output; r input; r_noise input
function r_mea = fcn(t,r,r_noise)


    if  t>30 && t<41
        r_mea = r_noise;
    else
        r_mea = r;
    end


end

== matlab function Y3Tiltrotor_sim3_INDI/Y3 Tiltrotor Aircraft Model/States Bus/MATLAB Function1 ==
  data: vxyz input; course output; gndSpeed output
function [course, gndSpeed] = fcn(vxyz)

vx = vxyz(1);
vy = vxyz(2);
course = atan2(vy, vx);
gndSpeed = norm([vx vy 0]);

== matlab function Y3Tiltrotor_sim3_INDI/Y3 Tiltrotor Aircraft Model/Subsystem/Aerodynamic Forces and Moments/Compute Body Frame Aerodynamic Forces and Moments/Wind frame F& M/Longitudinal Channel/CD/CD(alpha) ==
  data: alpha input; CD_alpha output
function CD_alpha = piecewise_CD_alpha(alpha)

    c1 = 10.5;
    c2 = 0.023013;
    c3 = 0.000398;
    c4 = 1.077953;
    c5 = -1.061505;
    c6 = 0.919668;
    c7 = -7.769775;
    c8 = 49.988;
    c9 = -0.043323;
    c10 = 1.088698;
    c11 = 0.891002;
    c12 = -9.586878;

    CD_alpha = zeros(size(alpha));

    idx_pos = alpha >= 0;
    if any(idx_pos)
        alpha_pos = alpha(idx_pos);
        CD_alpha(idx_pos) = (1+tanh(c1*(18.4^2-alpha_pos.^2)))/(1+tanh(c1*18.4^2)).*(c2+c3*alpha_pos.^2)...
            +(1-(1+tanh(c1*(18.4^2-alpha_pos.^2)))/(1+tanh(c1*18.4^2))).*(c4+c5*sin(c6*pi/180*alpha_pos+c7).^2);
    end
    
    idx_neg = alpha < 0;
    if any(idx_neg)
        alpha_neg = alpha(idx_neg);
        CD_alpha(idx_neg) = (1+tanh(c8*(15^2-alpha_neg.^2)))/(1+tanh(c8*15^2)).*(c2+c3*alpha_neg.^2)...
            +(1-(1+tanh(c8*(15^2-alpha_neg.^2)))/(1+tanh(c8*15^2))).*(c9+c10*sin(c11*pi/180*alpha_neg+c12).^2);
    end

end

== matlab function Y3Tiltrotor_sim3_INDI/Y3 Tiltrotor Aircraft Model/Subsystem/Aerodynamic Forces and Moments/Compute Body Frame Aerodynamic Forces and Moments/Wind frame F& M/Longitudinal Channel/Cm/Cm(alpha) ==
  data: Cm_alpha output; alpha input
function Cm_alpha = piecewise_Cm_alpha(alpha)

    c1 = 0.000219;
    c2 = -0.011442;
    c3 = 0.056866;
    c4 = -3.422369;
    c5 = -1.763366;
    c6 = -0.059447;
    c7 = 3.052526;
    c8 = 0.000256;
    c9 = -3.005585;
    c10 = -0.035985;
    c11 = -15.643618;

    Cm_alpha = zeros(size(alpha));

    idx_pos = alpha >= 0;
    if any(idx_pos)
        alpha_pos = alpha(idx_pos);
        Cm_alpha(idx_pos) = (1+tanh(c1*(18.4^2-alpha_pos.^2)))/(1+tanh(c1*18.4^2)).*(c2+c3*sin(c4*pi/180*alpha_pos))...
            +(1-(1+tanh(c1*(18.4^2-alpha_pos.^2)))/(1+tanh(c1*18.4^2))).*(c5*sin(c6*pi/180*alpha_pos+c7));
    end
    
    idx_neg = alpha < 0;
    if any(idx_neg)
        alpha_neg = alpha(idx_neg);
        Cm_alpha(idx_neg) = (1+tanh(c8*(15^2-alpha_neg.^2)))/(1+tanh(c8*15^2)).*(c2+c3*sin(c4*pi/180*alpha_neg))...
            +(1-(1+tanh(c8*(15^2-alpha_neg.^2)))/(1+tanh(c8*15^2))).*(c9*sin(c10*pi/180*alpha_neg+c11));
    end

end

== matlab function Y3Tiltrotor_sim3_INDI/Y3 Tiltrotor Aircraft Model/Subsystem/Aerodynamic Forces and Moments/Compute Body Frame Aerodynamic Forces and Moments/Wind frame F& M/Lateral Channel/CY/CY(beta) ==
  data: CY_beta output; beta input
function CY_beta = fcn_CY_beta(beta)

    c1 = 65.424349;
    c2 = 41.5;
    c3 = 0.100430;
    c4 = -1.744107;
    c5 = 0.083409;
    c6 = 1.914772;
    c7 = -3.141796;

    CY_beta = (1+tanh(c1*(c2^2-beta.^2)))/(1+tanh(c1*c2^2)).*(c3*sin(c4*pi/180*beta))...
        + (1-(1+tanh(c1*(c2^2-beta.^2)))/(1+tanh(c1*c2^2))).*(c5*sin(c6*pi/180*beta+c7));

end

== matlab function Y3Tiltrotor_sim3_INDI/Y3 Tiltrotor Aircraft Model/Subsystem/Aerodynamic Forces and Moments/Compute Body Frame Aerodynamic Forces and Moments/Wind frame F& M/Lateral Channel/Cl/Cl(beta) ==
  data: Cl1_beta output; beta input
function Cl1_beta = fcn_Cl1_beta(beta)

    c1 = 18.339628;
    c2 = 41.5;
    c3 = 0.035354;
    c4 = -1.788085;
    c5 = 0.035299;
    c6 = -1.515415;
    c7 = 0.001573;

    Cl1_beta = (1+tanh(c1*(c2^2-beta.^2)))/(1+tanh(c1*c2^2)).*(c3*sin(c4*pi/180*beta))...
        + (1-(1+tanh(c1*(c2^2-beta.^2)))/(1+tanh(c1*c2^2))).*(c5*sin(c6*pi/180*beta+c7));

end

== matlab function Y3Tiltrotor_sim3_INDI/Y3 Tiltrotor Aircraft Model/Subsystem/Aerodynamic Forces and Moments/Compute Body Frame Aerodynamic Forces and Moments/Wind frame F& M/Lateral Channel/Cn/Cn(beta) ==
  data: Cn_beta output; beta input
function Cn_beta = fcn_Cn_beta(beta)

    c1 = 16.018126;
    c2 = 41.5;
    c3 = 0.045296;
    c4 = 0.918923;
    c5 = 0.028417;
    c6 = 1.203453;
    c7 = 6.274968;

    Cn_beta = (1+tanh(c1*(c2^2-beta.^2)))/(1+tanh(c1*c2^2)).*(c3*sin(c4*pi/180*beta))...
        + (1-(1+tanh(c1*(c2^2-beta.^2)))/(1+tanh(c1*c2^2))).*(c5*sin(c6*pi/180*beta+c7));

end

== matlab function Y3Tiltrotor_sim3_INDI/Y3 Tiltrotor Aircraft Model/Subsystem/Aerodynamic Forces and Moments/Compute Body Frame Aerodynamic Forces and Moments/Wind frame F& M/Longitudinal Channel/Cm/Cm(delta_e) ==
  data: delta_e input; Cm_delta_e output
function Cm_delta_e = fcn_Cm_delta_e(delta_e)

    c1 = 0.000301;
    c2 = -1.724970;
    c3 = 0.142608;
    c4 = 0.109046;
    c5 = 0.694663;
    c6 = -2.968985;

    Cm_delta_e = (1+tanh(c1*(47.5^2-delta_e.^2)))/(1+tanh(c1*47.5^2)).*(c2*sin(c3*pi/180*delta_e))...
            +(1-(1+tanh(c1*(47.5^2-delta_e.^2)))/(1+tanh(c1*47.5^2))).*(c4*sin(c5*pi/180*delta_e+c6));

end
